simulink model "Synthetic_Signal_HAR"  (R2025a)
settings: Solver=VariableStepAuto  StartTime=0.0  StopTime=10.0  RelTol=1e-3
settings Model: Creator=vvsha  LastModifiedBy=vvsha

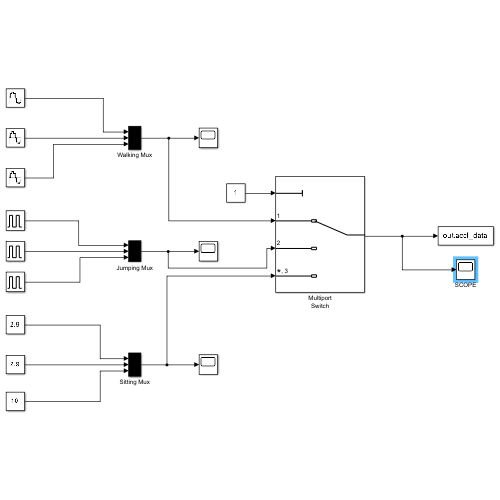
[thumbnail: Simulink's stored preview of the top-level diagram]
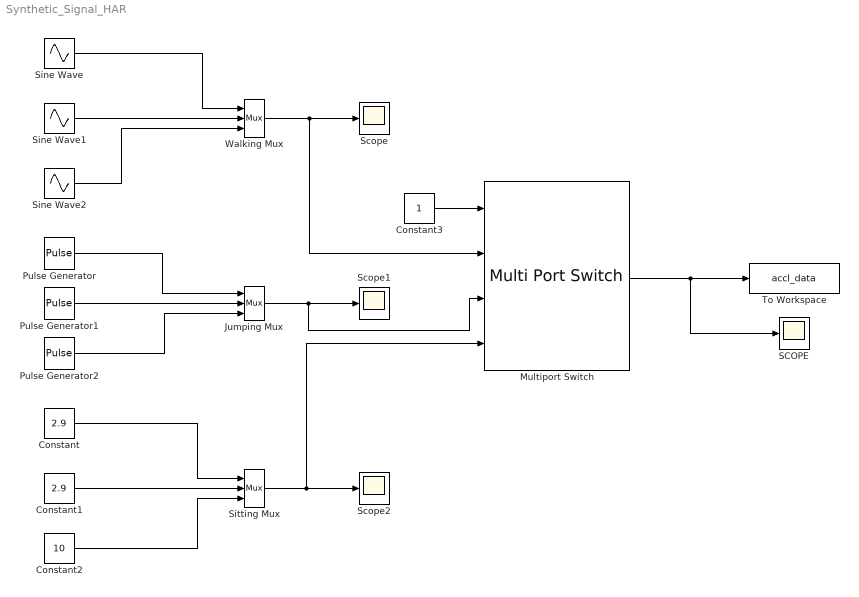
== system Synthetic_Signal_HAR ==
  Constant : Constant  Value=2.9  SampleTime=0.1
  Constant1 : Constant  Value=2.9  SampleTime=0.1
  Constant2 : Constant  Value=10  SampleTime=0.1
  Constant3 : Constant
  Jumping Mux : Mux  Inputs=3
  Multiport Switch : MultiPortSwitch  SaturateOnIntegerOverflow=off  InputSameDT=off
  Pulse Generator : DiscretePulseGenerator  PulseType=Time based  Amplitude=15  Period=1  PulseWidth=10
  Pulse Generator1 : DiscretePulseGenerator  PulseType=Time based  Amplitude=45  Period=1  PulseWidth=10
  Pulse Generator2 : DiscretePulseGenerator  PulseType=Time based  Amplitude=5  Period=1  PulseWidth=10
  SCOPE : Scope
      settings: ActiveDisplayYMinimum=-12.498603651397994  ActiveDisplayYMaximum=12.495107106172048  DataLoggingVariableName=ScopeData3
  Scope : Scope
      settings: ActiveDisplayYMinimum=-12.498603651397994  ActiveDisplayYMaximum=12.495107106172048
  Scope1 : Scope
      settings: ActiveDisplayYMinimum=-0.37499999999999989  ActiveDisplayYMaximum=3.375
  Scope2 : Scope
      settings: ActiveDisplayYMinimum=-0.37499999999999989  ActiveDisplayYMaximum=3.375  DataLoggingVariableName=ScopeData2
  Sine Wave : Sin  Amplitude=5  SampleTime=0.1
  Sine Wave1 : Sin  Amplitude=7  SampleTime=0.1
  Sine Wave2 : Sin  Amplitude=10  SampleTime=0.1
  Sitting Mux : Mux  Inputs=3
  To Workspace : ToWorkspace  VariableName=accl_data  SaveFormat=Timeseries  SampleTime=-1
  Walking Mux : Mux  Inputs=3
  wires:
  Sine Wave/1 -> Walking Mux/1
  Sine Wave2/1 -> Walking Mux/3
  Sine Wave1/1 -> Walking Mux/2
  Walking Mux/1 -> Multiport Switch/2, Scope/1
  Pulse Generator/1 -> Jumping Mux/1
  Pulse Generator1/1 -> Jumping Mux/2
  Pulse Generator2/1 -> Jumping Mux/3
  Jumping Mux/1 -> Scope1/1, Multiport Switch/3
  Constant/1 -> Sitting Mux/1
  Constant1/1 -> Sitting Mux/2
  Constant2/1 -> Sitting Mux/3
  Sitting Mux/1 -> Multiport Switch/4, Scope2/1
  Constant3/1 -> Multiport Switch/1
  Multiport Switch/1 -> SCOPE/1, To Workspace/1
